simulink model "hopper_6dof_NED_v2_ground"  (R2026a)
settings: Solver=ode3  StopTime=30  FixedStep=1e-3  RelTol=1e-5
undefined symbols (not defined in the file): cg_init, dcg_dMfu_table, dcg_dMox_table, dI_dMfu_table, dI_dMox_table, ENGINE, engine_cg, engine_mass, fu_axial_damping_ratios, fu_lateral_damping_ratios, fu_mass_profile, fu_masses, fu_mdot_data, g, h, IN, K1flat, K2grid, k_leg, m0, magnitude, MoI_init, mount_cg, OUT, ox_axial_damping_ratios, ox_lateral_damping_ratios, ox_mass_profile, ox_masses, ox_mdot_data, pressureLevels, tank_r, TANKS, Target_Trajectory, tgrid, thrust_data, unom, uwndTable, VEH, vwndTable
libraries: fl_lib x31, nesl_utility x25, matrix_library x18, SimscapeFluids_lib x10, simulink x9, simulink_extras x7, slpidlib x7, dspmathops x4, dspindex x3, sl_discontinuities x2, aerolibanim x1, commrandsrc3 x1
(part 7 of 7)

== system hopper_6dof_NED_v2_ground/Wind Forces/If Action Subsystem1 ==
  In1 : Inport
  Action Port : ActionPort  ActionPortLabel=elseif(u1 == 2)
  Constant : Constant  Value=IN.wind.uwind
  Constant1 : Constant  Value=IN.wind.vwind
  Constant3 : Constant  Value=[10;20]
  Mux : Mux  Inputs=2
  Terminator : Terminator
  Out2 : Outport
  wires:
  In1/1 -> Terminator/1
  Mux/1 -> Out2/1
  Constant/1 -> Mux/1
  Constant1/1 -> Mux/2

== system hopper_6dof_NED_v2_ground/Wind Forces/If Action Subsystem2 ==
  In1 : Inport
  Action Port : ActionPort  ActionPortLabel=else
  Display : Display
  Display1 : Display
  Latitude : Constant  Value=33.78
  Longitude : Constant  Value=84.40
  Month : Constant  Value=4
  Mux : Mux  Inputs=2
  Pressure (mb) : Constant  Value=1000
  Terminator : Terminator
  n-D Lookup Table : Lookup_n-D  NumberOfTableDimensions=4  BreakpointsForDimension1=1:12  BreakpointsForDimension2=pressureLevels  BreakpointsForDimension3=[32.5 35]  BreakpointsForDimension4=[82.5 85]  Table=uwndTable  ExtrapMethod=Clip  InternalRulePriority=Speed  RndMeth=Simplest
      settings: InputPortMap=u0,u1,u2,u3
  n-D Lookup Table1 : Lookup_n-D  NumberOfTableDimensions=4  BreakpointsForDimension1=1:12  BreakpointsForDimension2=pressureLevels  BreakpointsForDimension3=[32.5 35]  BreakpointsForDimension4=[82.5 85]  Table=vwndTable  InternalRulePriority=Speed  RndMeth=Simplest
      settings: InputPortMap=u0,u1,u2,u3
  Out1 : Outport
  wires:
  Month/1 -> n-D Lookup Table1/1, n-D Lookup Table/1
  Pressure (mb)/1 -> n-D Lookup Table1/2, n-D Lookup Table/2
  Latitude/1 -> n-D Lookup Table1/3, n-D Lookup Table/3
  In1/1 -> Terminator/1
  Longitude/1 -> n-D Lookup Table1/4, n-D Lookup Table/4
  n-D Lookup Table/1 -> Display/1, Mux/1
  n-D Lookup Table1/1 -> Display1/1, Mux/2
  Mux/1 -> Out1/1

== system hopper_6dof_NED_v2_ground/Fluid Network2/COPV/COPV Leakage ==
  Leak Rate : fl_lib/Gas/Elements/Flow Resistance (G)  delta_p_nominal=0.001 MPa  mdot_nominal=0.0000000001 kg/s  rho_nominal=0 kg/m^3  area=0.01 m^2  laminar_fraction=1e-3
  Mass & Energy Flow Rate Sensor (G)2 : fl_lib/Gas/Sensors/Flow Rate Sensor (G)  mass_flow_measure=true  volumetric_flow_measure=false  volumetric_flow_conditions=foundation.enum.volumetric_flow_conditions.actual  p_std=0.101325 MPa  T_std=20 degC  energy_flow_measure=true
  PS-Simulink Converter7 : nesl_utility/PS-Simulink Converter  PhysicalDomain=network_engine_domain  SubClassName=ps_output  LeftPortType=input  RightPortType=output  PseudoPeriodic=off  Frequencies=[]  VectorFormat=inherit  Unit=inherit  AffineConversion=off
  Pressurant Mass Leak Rate : Scope  Commented=on
      settings: ActiveDisplayYMinimum=-1  ActiveDisplayYMaximum=1
  Reservoir (G) : fl_lib/Gas/Elements/Reservoir (G)  pressure_input=false  pressure_spec=foundation.enum.pressure_spec.atmospheric  reservoir_pressure=0.101325 MPa  temperature_input=false  reservoir_temperature=293.15 K  area_A=0.01 m^2  input_error_spec=foundation.enum.input_range_error.warn
  Conn1 : PMIOPort  Side=Right
  wires:
  PS-Simulink Converter7/1 -> Pressurant Mass Leak Rate/1
  connections:
  Conn1/RConn1 -- Leak Rate/RConn1
  Leak Rate/LConn1 -- Mass & Energy Flow Rate Sensor (G)2/LConn1
  Mass & Energy Flow Rate Sensor (G)2/RConn1 -- Reservoir (G)/LConn1
  Mass & Energy Flow Rate Sensor (G)2/RConn2 -- PS-Simulink Converter7/LConn1

== system hopper_6dof_NED_v2_ground/Ground1/Ground Interaction 1/If Action Subsystem ==
  Velocity : Inport
  Action Port : ActionPort
  Fg : Constant  Value=m0 * IN.const.g0
  Gain : Gain  Gain=-1
  Normalization : dspmathops/Normalization  NormType=Squared 2-norm  Bias=1e-10  NormOver=Each column  Dimension=1  roundingMode=Floor  overflowMode=off  accumDataTypeStr=Inherit: Same as product output  accumLastDataTypeStr=Inherit: Same as product output  outputDataTypeStr=Inherit: Same as product output  outputMin=[]  outputMax=[]  outputLastDataTypeStr=Inherit: Same as product output
  Product : Product  Inputs=3
  mu : Constant  Value=0.6
  Fk : Outport
  wires:
  Velocity/1 -> Normalization/1
  Normalization/1 -> Product/1
  Fg/1 -> Product/2
  mu/1 -> Product/3
  Product/1 -> Gain/1
  Gain/1 -> Fk/1

== system hopper_6dof_NED_v2_ground/Ground1/Ground Interaction 1/If Action Subsystem1 ==
  Action Port : ActionPort
  Zero : Constant  Value=[0 0 0]  OutDataTypeStr=Inherit: Inherit via back propagation
  Out1 : Outport
  wires:
  Zero/1 -> Out1/1

== system hopper_6dof_NED_v2_ground/Ground1/Ground Interaction 2/If Action Subsystem ==
  Velocity : Inport
  Action Port : ActionPort
  Fg : Constant  Value=m0 * IN.const.g0
  Gain : Gain  Gain=-1
  Normalization : dspmathops/Normalization  NormType=Squared 2-norm  Bias=1e-10  NormOver=Each column  Dimension=1  roundingMode=Floor  overflowMode=off  accumDataTypeStr=Inherit: Same as product output  accumLastDataTypeStr=Inherit: Same as product output  outputDataTypeStr=Inherit: Same as product output  outputMin=[]  outputMax=[]  outputLastDataTypeStr=Inherit: Same as product output
  Product : Product  Inputs=3
  mu : Constant  Value=0.6
  Fk : Outport
  wires:
  Velocity/1 -> Normalization/1
  Normalization/1 -> Product/1
  Fg/1 -> Product/2
  mu/1 -> Product/3
  Product/1 -> Gain/1
  Gain/1 -> Fk/1

== system hopper_6dof_NED_v2_ground/Ground1/Ground Interaction 2/If Action Subsystem1 ==
  Action Port : ActionPort
  Zero : Constant  Value=[0 0 0]  OutDataTypeStr=Inherit: Inherit via back propagation
  Out1 : Outport
  wires:
  Zero/1 -> Out1/1

== system hopper_6dof_NED_v2_ground/Ground1/Ground Interaction 3/If Action Subsystem ==
  Velocity : Inport
  Action Port : ActionPort
  Fg : Constant  Value=m0 * IN.const.g0
  Gain : Gain  Gain=-1
  Normalization : dspmathops/Normalization  NormType=Squared 2-norm  Bias=1e-10  NormOver=Each column  Dimension=1  roundingMode=Floor  overflowMode=off  accumDataTypeStr=Inherit: Same as product output  accumLastDataTypeStr=Inherit: Same as product output  outputDataTypeStr=Inherit: Same as product output  outputMin=[]  outputMax=[]  outputLastDataTypeStr=Inherit: Same as product output
  Product : Product  Inputs=3
  mu : Constant  Value=0.6
  Fk : Outport
  wires:
  Velocity/1 -> Normalization/1
  Normalization/1 -> Product/1
  Fg/1 -> Product/2
  mu/1 -> Product/3
  Product/1 -> Gain/1
  Gain/1 -> Fk/1

== system hopper_6dof_NED_v2_ground/Ground1/Ground Interaction 3/If Action Subsystem1 ==
  Action Port : ActionPort
  Zero : Constant  Value=[0 0 0]  OutDataTypeStr=Inherit: Inherit via back propagation
  Out1 : Outport
  wires:
  Zero/1 -> Out1/1

== system hopper_6dof_NED_v2_ground/Ground1/Ground Interaction 4/If Action Subsystem ==
  Velocity : Inport
  Action Port : ActionPort
  Fg : Constant  Value=m0 * IN.const.g0
  Gain : Gain  Gain=-1
  Normalization : dspmathops/Normalization  NormType=Squared 2-norm  Bias=1e-10  NormOver=Each column  Dimension=1  roundingMode=Floor  overflowMode=off  accumDataTypeStr=Inherit: Same as product output  accumLastDataTypeStr=Inherit: Same as product output  outputDataTypeStr=Inherit: Same as product output  outputMin=[]  outputMax=[]  outputLastDataTypeStr=Inherit: Same as product output
  Product : Product  Inputs=3
  mu : Constant  Value=0.6
  Fk : Outport
  wires:
  Velocity/1 -> Normalization/1
  Normalization/1 -> Product/1
  Fg/1 -> Product/2
  mu/1 -> Product/3
  Product/1 -> Gain/1
  Gain/1 -> Fk/1

== system hopper_6dof_NED_v2_ground/Ground1/Ground Interaction 4/If Action Subsystem1 ==
  Action Port : ActionPort
  Zero : Constant  Value=[0 0 0]  OutDataTypeStr=Inherit: Inherit via back propagation
  Out1 : Outport
  wires:
  Zero/1 -> Out1/1

== matlab function hopper_6dof_NED_v2_ground/Slosh/Oxidizer Yaw Force/MATLAB Function ==
  data: ox_yaw_accel input; accel_term output; ox_lateral_pendulum_l input
function accel_term = fcn(ox_yaw_accel, ox_lateral_pendulum_l)

accel_term = -ox_yaw_accel / ox_lateral_pendulum_l;

end

== matlab function hopper_6dof_NED_v2_ground/Slosh/Oxidizer Yaw Force/MATLAB Function1 ==
  data: ox_yaw_phi input; ang_term output; ox_lateral_natural_freq input
function ang_term = fcn(ox_yaw_phi, ox_lateral_natural_freq)

ang_term = -ox_lateral_natural_freq^2 * ox_yaw_phi;

end

== matlab function hopper_6dof_NED_v2_ground/Slosh/Oxidizer Yaw Force/MATLAB Function2 ==
  data: ox_yaw_phi_dot input; velo_term output; ox_lateral_natural_freq input; ox_lateral_damping input
function velo_term = fcn(ox_yaw_phi_dot, ox_lateral_natural_freq,ox_lateral_damping)

velo_term = -2 * ox_lateral_damping * ox_lateral_natural_freq * ox_yaw_phi_dot;
end

== matlab function hopper_6dof_NED_v2_ground/Slosh/Oxidizer Yaw Force/MATLAB Function3 ==
  data: ox_yaw_phi_ddot input; ox_yaw_f output; ox_lateral_slosh_mass input; ox_lateral_pendulum_l input
function ox_yaw_f = fcn(ox_yaw_phi_ddot, ox_lateral_slosh_mass, ox_lateral_pendulum_l)

ox_yaw_f = ox_lateral_slosh_mass * ox_lateral_pendulum_l * ox_yaw_phi_ddot;
end

== matlab function hopper_6dof_NED_v2_ground/Slosh/Oxidizer Axial Force/MATLAB Function ==
  data: ox_axial_accel input; accel_term output; ox_axial_pendulum_l input
function accel_term = fcn(ox_axial_accel, ox_axial_pendulum_l)

accel_term = -ox_axial_accel / ox_axial_pendulum_l;

end

== matlab function hopper_6dof_NED_v2_ground/Slosh/Oxidizer Axial Force/MATLAB Function1 ==
  data: ox_axial_phi input; ang_term output; ox_axial_natural_freq input
function ang_term = fcn(ox_axial_phi, ox_axial_natural_freq)

ang_term = -ox_axial_natural_freq^2 * ox_axial_phi;

end

== matlab function hopper_6dof_NED_v2_ground/Slosh/Oxidizer Axial Force/MATLAB Function2 ==
  data: ox_axial_phi_dot input; velo_term output; ox_axial_natural_freq input; ox_axial_damping input
function velo_term = fcn(ox_axial_phi_dot, ox_axial_natural_freq,ox_axial_damping)

velo_term = -2 * ox_axial_damping * ox_axial_natural_freq * ox_axial_phi_dot;
end

== matlab function hopper_6dof_NED_v2_ground/Slosh/Oxidizer Axial Force/MATLAB Function3 ==
  data: ox_axial_phi_ddot input; ox_axial_f output; ox_axial_slosh_mass input; ox_axial_pendulum_l input
function ox_axial_f = fcn(ox_axial_phi_ddot, ox_axial_slosh_mass, ox_axial_pendulum_l)

ox_axial_f = ox_axial_slosh_mass * ox_axial_pendulum_l * ox_axial_phi_ddot;
end

== matlab function hopper_6dof_NED_v2_ground/Slosh/Fuel Axial Force/MATLAB Function ==
  data: fu_axial_accel input; accel_term output; fu_axial_pendulum_l input
function accel_term = fcn(fu_axial_accel, fu_axial_pendulum_l)

accel_term = -fu_axial_accel / fu_axial_pendulum_l;

end

== matlab function hopper_6dof_NED_v2_ground/Slosh/Fuel Axial Force/MATLAB Function1 ==
  data: fu_axial_phi input; ang_term output; fu_axial_natural_freq input
function ang_term = fcn(fu_axial_phi, fu_axial_natural_freq)

ang_term = -fu_axial_natural_freq^2 * fu_axial_phi;

end

== matlab function hopper_6dof_NED_v2_ground/Slosh/Fuel Axial Force/MATLAB Function2 ==
  data: fu_axial_phi_dot input; velo_term output; fu_axial_natural_freq input; fu_axial_damping input
function velo_term = fcn(fu_axial_phi_dot, fu_axial_natural_freq,fu_axial_damping)

velo_term = -2 * fu_axial_damping * fu_axial_natural_freq * fu_axial_phi_dot;
end

== matlab function hopper_6dof_NED_v2_ground/Slosh/Fuel Axial Force/MATLAB Function3 ==
  data: fu_axial_phi_ddot input; fu_axial_f output; fu_axial_slosh_mass input; fu_axial_pendulum_l input
function fu_axial_f = fcn(fu_axial_phi_ddot, fu_axial_slosh_mass, fu_axial_pendulum_l)

fu_axial_f = fu_axial_slosh_mass * fu_axial_pendulum_l * fu_axial_phi_ddot;
end

== matlab function hopper_6dof_NED_v2_ground/Slosh/Fuel Yaw Force/MATLAB Function ==
  data: fu_pitch_accel input; accel_term output; fu_lateral_pendulum_l input
function accel_term = fcn(fu_pitch_accel, fu_lateral_pendulum_l)

accel_term = -fu_pitch_accel / fu_lateral_pendulum_l;

end

== matlab function hopper_6dof_NED_v2_ground/Slosh/Fuel Yaw Force/MATLAB Function1 ==
  data: fu_pitch_phi input; ang_term output; fu_lateral_natural_freq input
function ang_term = fcn(fu_pitch_phi, fu_lateral_natural_freq)

ang_term = -fu_lateral_natural_freq^2 * fu_pitch_phi;

end

== matlab function hopper_6dof_NED_v2_ground/Slosh/Fuel Yaw Force/MATLAB Function2 ==
  data: fu_pitch_phi_dot input; velo_term output; fu_lateral_natural_freq input; fu_lateral_damping input
function velo_term = fcn(fu_pitch_phi_dot, fu_lateral_natural_freq,fu_lateral_damping)

velo_term = -2 * fu_lateral_damping * fu_lateral_natural_freq * fu_pitch_phi_dot;
end

== matlab function hopper_6dof_NED_v2_ground/Slosh/Fuel Yaw Force/MATLAB Function3 ==
  data: fu_pitch_phi_ddot input; fu_pitch_f output; fu_lateral_slosh_mass input; fu_lateral_pendulum_l input
function fu_pitch_f = fcn(fu_pitch_phi_ddot, fu_lateral_slosh_mass, fu_lateral_pendulum_l)

fu_pitch_f = fu_lateral_slosh_mass * fu_lateral_pendulum_l * fu_pitch_phi_ddot;
end

== matlab function hopper_6dof_NED_v2_ground/Slosh/Fuel Pitch Force/MATLAB Function ==
  data: fu_yaw_accel input; accel_term output; fu_lateral_pendulum_l input
function accel_term = fcn(fu_yaw_accel, fu_lateral_pendulum_l)

accel_term = -fu_yaw_accel / fu_lateral_pendulum_l;

end

== matlab function hopper_6dof_NED_v2_ground/Slosh/MATLAB Function ==
  data: ox_lateral_natural_freq output; ox_axial_natural_freq output; ox_mass input; ox_lateral_slosh_mass output; ox_axial_slosh_mass output; ox_lateral_pendulum_l output; ox_aeff input; ox_axial_pendulum_l output; ox_lateral_damping output; ox_axial_damping output; tank_r input; ox_lateral_damping input; ox_axial_damping input
function [ox_lateral_natural_freq, ox_axial_natural_freq, ox_lateral_slosh_mass,ox_axial_slosh_mass, ox_lateral_pendulum_l, ox_axial_pendulum_l, ox_lateral_damping, ox_axial_damping]  = slosh_parameters(ox_mass, ox_aeff, tank_r, ox_lateral_damping, ox_axial_damping)

zeta = 1.841; % 1st eigen mode of oscillation for a cylindrical tank
ox_density = 1141;   % kg/m^3
% ox_tank_cg = 1.854; % m
% ox_tank_h =  TANKS.singular.oxidizer.h;
geff = norm(ox_aeff) + 0.001;

% Oxidizer Fluid
if ox_mass > 0.001
   h_ox_fluid = (ox_mass / ox_density) / (pi * tank_r^2);

   % Slosh Natural Frequencies
    ox_lateral_natural_freq = sqrt(zeta * geff / tank_r) * tanh(zeta * h_ox_fluid / tank_r);
    ox_axial_natural_freq = pi * sqrt(geff / h_ox_fluid);

    % Slosh Masses 
    ox_lateral_slosh_mass = ox_mass * (2 * tank_r * tanh(2 * zeta * h_ox_fluid / (2 * tank_r))) / (zeta * (zeta^2 - 1) * h_ox_fluid);
    ox_axial_slosh_mass = 1 / (pi^2) *  ox_mass;

    % Slosh Pendulum Lengths
    ox_lateral_pendulum_l = (2 * tank_r) / (2 * zeta * tanh(2*zeta * h_ox_fluid / (2 * tank_r)));
    ox_axial_pendulum_l = geff / ox_axial_natural_freq^2;
else
   h_ox_fluid = 0; 
   ox_lateral_natural_freq = 0;
   ox_axial_natural_freq = 0;
   ox_lateral_slosh_mass = 0;
   ox_axial_slosh_mass = 0;
   ox_lateral_pendulum_l = 1;
   ox_axial_pendulum_l = 1;
end



end

== matlab function hopper_6dof_NED_v2_ground/Slosh/Fuel Pitch Force/MATLAB Function1 ==
  data: fu_yaw_phi input; ang_term output; fu_lateral_natural_freq input
function ang_term = fcn(fu_yaw_phi, fu_lateral_natural_freq)

ang_term = -fu_lateral_natural_freq^2 * fu_yaw_phi;

end

== matlab function hopper_6dof_NED_v2_ground/Slosh/Fuel Pitch Force/MATLAB Function2 ==
  data: fu_yaw_phi_dot input; velo_term output; fu_lateral_natural_freq input; fu_lateral_damping input
function velo_term = fcn(fu_yaw_phi_dot, fu_lateral_natural_freq, fu_lateral_damping)

velo_term = -2 * fu_lateral_damping * fu_lateral_natural_freq * fu_yaw_phi_dot;
end

== matlab function hopper_6dof_NED_v2_ground/Slosh/Fuel Pitch Force/MATLAB Function3 ==
  data: fu_yaw_phi_ddot input; fu_yaw_f output; fu_lateral_slosh_mass input; fu_lateral_pendulum_l input
function fu_yaw_f = fcn(fu_yaw_phi_ddot, fu_lateral_slosh_mass, fu_lateral_pendulum_l)

fu_yaw_f = fu_lateral_slosh_mass * fu_lateral_pendulum_l * fu_yaw_phi_ddot;
end

== matlab function hopper_6dof_NED_v2_ground/CG // MOI Script v3/MATLAB Function ==
  data: r_ox input; I_m_ox output
function I_m_ox = fcn(r_ox)
x = r_ox(1);
y = r_ox(2);
z = r_ox(3);

I_m_ox = [y^2 + z^2 -x*y x*z;
       -x*y x^2 + z^2 -y*z;
       -x*z y*z  x^2 + y^2
    ];

== matlab function hopper_6dof_NED_v2_ground/CG // MOI Script v3/MATLAB Function1 ==
  data: r_fu input; I_m_fu output
function I_m_fu = fcn(r_fu)
x = r_fu(1);
y = r_fu(2);
z = r_fu(3);

I_m_fu = [y^2 + z^2 -x*y x*z;
       -x*y x^2 + z^2 -y*z;
       -x*z y*z  x^2 + y^2
    ];

== matlab function hopper_6dof_NED_v2_ground/Slosh/Oxidizer Axial Force/MATLAB Function4 ==
  data: x_omega_dot input; x_slosh_torque output; ox_axial_slosh_mass input; ox_axial_pendulum_l input; slosh_angular_accel input
function x_slosh_torque = fcn(x_omega_dot, ox_axial_slosh_mass, ox_axial_pendulum_l, slosh_angular_accel)

I_s = ox_axial_slosh_mass * ox_axial_pendulum_l^2;

x_slosh_torque = -I_s*(x_omega_dot - slosh_angular_accel);

== matlab function hopper_6dof_NED_v2_ground/Slosh/Fuel Axial Force/MATLAB Function4 ==
  data: x_omega_dot input; x_slosh_torque output; fu_axial_slosh_mass input; fu_axial_pendulum_l input; slosh_angular_accel input
function x_slosh_torque = fcn(x_omega_dot, fu_axial_slosh_mass, fu_axial_pendulum_l, slosh_angular_accel)

I_s = fu_axial_slosh_mass * fu_axial_pendulum_l^2;

x_slosh_torque = -I_s*(x_omega_dot - slosh_angular_accel);

== matlab function hopper_6dof_NED_v2_ground/Slosh/Oxidizer Yaw Force/MATLAB Function4 ==
  data: y_omega_dot input; y_slosh_torque output; ox_lateral_slosh_mass input; ox_lateral_pendulum_l input; slosh_angular_accel input
function y_slosh_torque = fcn(y_omega_dot, ox_lateral_slosh_mass, ox_lateral_pendulum_l, slosh_angular_accel)

I_s = ox_lateral_slosh_mass * ox_lateral_pendulum_l^2;

y_slosh_torque = -I_s*(y_omega_dot - slosh_angular_accel);

== matlab function hopper_6dof_NED_v2_ground/Slosh/Fuel Yaw Force/MATLAB Function4 ==
  data: y_omega_dot input; y_slosh_torque output; fu_lateral_slosh_mass input; fu_lateral_pendulum_l input; slosh_angular_accel input
function y_slosh_torque = fcn(y_omega_dot, fu_lateral_slosh_mass, fu_lateral_pendulum_l, slosh_angular_accel)

I_s = fu_lateral_slosh_mass * fu_lateral_pendulum_l^2;

y_slosh_torque = -I_s*(y_omega_dot - slosh_angular_accel);

== matlab function hopper_6dof_NED_v2_ground/Slosh/Oxidizer Pitch Force/MATLAB Function4 ==
  data: z_omega_dot input; z_slosh_torque output; ox_lateral_slosh_mass input; ox_lateral_pendulum_l input; slosh_angular_accel input
function z_slosh_torque = fcn(z_omega_dot, ox_lateral_slosh_mass, ox_lateral_pendulum_l, slosh_angular_accel)

I_s = ox_lateral_slosh_mass * ox_lateral_pendulum_l^2;

z_slosh_torque = -I_s*(z_omega_dot - slosh_angular_accel);

== matlab function hopper_6dof_NED_v2_ground/Slosh/Fuel Pitch Force/MATLAB Function4 ==
  data: z_omega_dot input; z_slosh_torque output; fu_lateral_slosh_mass input; fu_lateral_pendulum_l input; slosh_angular_accel input
function z_slosh_torque = fcn(z_omega_dot, fu_lateral_slosh_mass, fu_lateral_pendulum_l, slosh_angular_accel)

I_s = fu_lateral_slosh_mass * fu_lateral_pendulum_l^2;

z_slosh_torque = -I_s*(z_omega_dot - slosh_angular_accel);

== matlab function hopper_6dof_NED_v2_ground/CG // MOI Script v3/MATLAB Function2 ==
  data: delta_y input; rot_mat output; delta_z input
function rot_mat = fcn(delta_y, delta_z)

rot_mat = [0 -delta_z delta_y;
           delta_z 0 0;
           -delta_y 0 0];

== matlab function hopper_6dof_NED_v2_ground/Fluid Network2/Fuel Throttle Valve Controller/Feed Forward ==
  data: mdot input; theta output; ptank input; pset input; rho input; CdA output
function [theta, CdA] = feed_forward(mdot,ptank,pset,rho)

dp = max(ptank - pset, 1e-6); % divide by zero error
CdA = mdot / sqrt(2*dp*rho);

CdA = max(CdA, 1e-7); % divide by zero error
Cv_vector = [1e-8, 0.01, 0.06, 0.21, 0.46, 0.83, 1.35, 2.04, 2.93];
CdA_vector = Cv_vector ./ 37.97;
theta_vector = 0.9.*[20,30,40,50,60,70,80,90,100];

theta = interp1(CdA_vector, theta_vector, CdA);
theta = min(theta, 90);
theta = max(theta, 0);
end

== matlab function hopper_6dof_NED_v2_ground/Fluid Network2/Fuel Throttle Valve Controller/MATLAB Function5 ==
  data: time input; rate_limit_up output; rate_limit_down output
function [rate_limit_up, rate_limit_down] = fcn(time)
if time < 0.5
    rate_limit_up = 1350;
else
    rate_limit_up = 40;
end
rate_limit_down = -rate_limit_up;

== matlab function hopper_6dof_NED_v2_ground/Fluid Network2/Fuel Throttle Valve Controller/System ==
  data: Ptank input; CdA input; mdot input; Pout output; rho input; dp output
function [Pout,dp] = theta_to_pressure(Ptank,CdA,mdot, rho)

% CdA = mdot/(sqrt((2*(ptank-pout)*rho)

%CdA = max(CdA, 1e-7);
dp = (mdot/CdA)^2*1/(2*rho);

% (mdot/CdA)^2*rho/2 is solving for the pout from the dp in CdA eqn
Pout = Ptank - dp;
Pout = max(Pout, 0);

== matlab function hopper_6dof_NED_v2_ground/Fluid Network2/MATLAB Function ==
  data: mdot_ox input; mdot_fuel input; eta_cstar input; Cf input; thrust output; Pc output; MR output; cstar_ideal input
function [thrust, Pc, MR] = engine_model(mdot_ox, mdot_fuel, eta_cstar, Cf, cstar_ideal)
%#codegen
% ENGINE_MODEL
%
% Inputs:
%   mdot_ox      - oxidizer mass flow rate [kg/s]
%   mdot_fuel    - fuel mass flow rate [kg/s]
%   eta_cstar    - c* efficiency [-]
%   Cf           - thrust coefficient [-]
%
% Outputs:
%   thrust       - thrust [N]
%   Pc           - chamber pressure [Pa]
%   MR           - mixture ratio [-]

    %% -------------------------
    % CONSTANTS
    % -------------------------
    At = 0.0008271;      % throat area [m^2]

    %% -------------------------
    % 1. Total mass flow
    % -------------------------
    mdot = mdot_ox + mdot_fuel;

    %% -------------------------
    % 2. Mixture ratio
    % -------------------------
    if mdot_fuel > 0
        MR = mdot_ox / mdot_fuel;
    else
        MR = 0; % avoid divide by zero
    end

    %% -------------------------
    % 3. Actual c*
    % -------------------------
    cstar_actual = eta_cstar * cstar_ideal;

    %% -------------------------
    % 4. Chamber pressure
    % -------------------------
    Pc = (mdot * cstar_actual) / At;

    %% -------------------------
    % 6. Thrust
    % -------------------------
    thrust = Cf * Pc * At;

    % Equivalent:
    % thrust = Cf * mdot * cstar_actual;

end

== matlab function hopper_6dof_NED_v2_ground/Fluid Network2/Ox Throttle Valve Controller/Feed Forward ==
  data: mdot input; theta output; ptank input; pset input; rho input; CdA output
function [theta, CdA] = feed_forward(mdot,ptank,pset,rho)

dp = max(ptank - pset, 1e-6); % divide by zero error
CdA = mdot / sqrt(2*dp*rho);

CdA = max(CdA, 1e-7); % divide by zero error
Cv_vector = [1e-8, 0.01, 0.06, 0.21, 0.46, 0.83, 1.35, 2.04, 2.93];
CdA_vector = Cv_vector ./ 37.97;
theta_vector = 0.9.*[20,30,40,50,60,70,80,90,100];

theta = interp1(CdA_vector, theta_vector, CdA);
theta = min(theta, 90);
theta = max(theta, 0);
end

== matlab function hopper_6dof_NED_v2_ground/Fluid Network2/Ox Throttle Valve Controller/MATLAB Function5 ==
  data: time input; rate_limit_up output; rate_limit_down output
function [rate_limit_up, rate_limit_down] = fcn(time)
if time < 0.5
    rate_limit_up = 1350;
else
    rate_limit_up = 40;
end
rate_limit_down = -rate_limit_up;

== matlab function hopper_6dof_NED_v2_ground/Fluid Network2/Ox Throttle Valve Controller/System ==
  data: Ptank input; CdA input; mdot input; Pout output; rho input; dp output
function [Pout,dp] = theta_to_pressure(Ptank,CdA,mdot, rho)

% CdA = mdot/(sqrt((2*(ptank-pout)*rho)

%CdA = max(CdA, 1e-7);
dp = (mdot/CdA)^2*1/(2*rho);

% (mdot/CdA)^2*rho/2 is solving for the pout from the dp in CdA eqn
Pout = Ptank - dp;
Pout = max(Pout, 0);

== matlab function hopper_6dof_NED_v2_ground/MATLAB Function ==
  data: t input; u output; x input; tgrid input; xref input; K1flat input; K2grid input; unom input
function u = Gain_Selector(t, x, tgrid, xref, K1flat, K2grid, unom)
%#codegen
% Fixed-size output: u is always 4x1

u = zeros(4,1);

x = x(:);              % should be 13x1 for 6DOF
N = length(tgrid);

% --- Clamp time and compute interval index ---
if t <= tgrid(1)
    idx = 1;
    w = 0.0;
elseif t >= tgrid(end)
    idx = N-1;
    w = 1.0;
else
    idx = 1;
    for k = 1:(N-1)
        if tgrid(k) <= t && t < tgrid(k+1)
            idx = k;
            break;
        end
    end
    t1 = tgrid(idx);
    t2 = tgrid(idx+1);
    w  = (t - t1) / (t2 - t1);
end

% --- Interpolate reference state (13x1) ---
xref_t = (1-w)*xref(idx,:)' + w*xref(idx+1,:)';

% --- Interpolate K1flat then reshape to 4x13 ---
Kflat = (1-w)*K1flat(idx,:) + w*K1flat(idx+1,:);
K1 = reshape(Kflat, 13, 4)';   % 4x13   (requires K1flat is N×52)

% --- Interpolate K2 (4x1) ---
K2 = (1-w)*K2grid(idx,:)' + w*K2grid(idx+1,:)';

% --- Interpolate nominal control (4x1) ---
u_nom = (1-w)*unom(idx,:)' + w*unom(idx+1,:)';

q     = x(10:13);
qref  = xref_t(10:13);

if dot(q,qref) < 0
    q = -q;
end

x_used = x;
x_used(10:13) = q;

dx = x_used - xref_t;


% --- Control law ---
%dx = (x - xref_t);          % 13x1
u  =u_nom+(-K1*dx)-K2;  
%fix

end

== matlab function hopper_6dof_NED_v2_ground/Fluid Network2/Thrust Commanded to mdot + bunch of other bs ==
  data: mdot_fuel output; rho_fuel_eng output; pc output; F_cmd input; rho_ox input; rho_fuel input; rho_ox_eng output; mdot_ox output; Cf input; MR input; cstar_ideal input; cstar_eff input
function [mdot_fuel, rho_fuel_eng, pc, rho_ox_eng, mdot_ox] = thrust_to_mdot( ...
   F_cmd, rho_ox, rho_fuel, Cf, MR, cstar_ideal, cstar_eff)
%#codegen
% Convert commanded thrust into mdots and convert densities to English units
%
% Outputs:
%   mdot_ox        - oxidizer mass flow rate [kg/s]
%   mdot_fuel      - fuel mass flow rate [kg/s]
%   rho_ox_eng     - oxidizer density [lb/ft^3]
%   rho_fuel_eng   - fuel density [lb/ft^3]
%   mdot_ox_lb     - oxidizer mass flow rate [lb/s]
%   mdot_fuel_lb   - fuel mass flow rate [lb/s]

    cstar = cstar_ideal * cstar_eff;
    At = 0.0008271;      % throat area [m^2]

    %% ---- DEFAULT OUTPUTS ----
    mdot_ox = 0;
    mdot_fuel = 0;
    rho_ox_eng = 0;
    rho_fuel_eng = 0;
    mdot_ox_lb = 0;
    mdot_fuel_lb = 0;

    %% ---- UNIT CONVERSION ----
    kgm3_to_lbft3 = 0.062428;
    kg_to_lb = 2.20462;

    rho_ox_eng = rho_ox * kgm3_to_lbft3;
    rho_fuel_eng = rho_fuel * kgm3_to_lbft3;

    %% ---- EFFECTIVE EXHAUST VELOCITY ----
    ve = Cf * cstar;


    %% ---- TOTAL MASS FLOW ----
    mdot_total = F_cmd / ve;

    pc = mdot_total * cstar / At;

    pc = pc * 0.000145038;

    %% ---- SPLIT BY MR ----
    mdot_ox = mdot_total * MR / (1 + MR);
    mdot_fuel = mdot_total / (1 + MR);


end

== matlab function hopper_6dof_NED_v2_ground/Slosh/MATLAB Function1 ==
  data: fu_mass input; fu_lateral_natural_freq output; fu_axial_natural_freq output; fu_lateral_slosh_mass output; fu_aeff input; fu_axial_slosh_mass output; fu_lateral_pendulum_l output; fu_axial_pendulum_l output; fu_lateral_damping output; fu_axial_damping output; tank_r input; fu_lateral_damping input; fu_axial_damping input
function [fu_lateral_natural_freq, fu_axial_natural_freq, fu_lateral_slosh_mass, fu_axial_slosh_mass, fu_lateral_pendulum_l, fu_axial_pendulum_l, fu_lateral_damping, fu_axial_damping]  = slosh_parameters(fu_mass, fu_aeff, tank_r, fu_lateral_damping, fu_axial_damping) 
zeta = 1.841; % 1st eigen mode of oscillation for a cylindrical tank
fu_density = 800;    % kg/m^3
% fu_tank_cg = 1.0668; % m
% fu_tank_h = TANKS.singular.fuel.h;
geff = norm(fu_aeff) + 0.001;

if fu_mass > 0.001
   h_fu_fluid = (fu_mass / fu_density) / (pi * tank_r^2);
   % Fluid sits at the bottom of the tank shell
   % z_fu_fluid = (fu_tank_cg - fu_tank_h/2) + (h_fu_fluid / 2);

   % Slosh Natural Frequencies
    fu_lateral_natural_freq = sqrt(zeta * geff / tank_r) * tanh(zeta * h_fu_fluid / tank_r);
    fu_axial_natural_freq = pi * sqrt(geff / h_fu_fluid);

    % Slosh Masses 
    fu_lateral_slosh_mass = fu_mass * (2 * tank_r * tanh(2 * zeta * h_fu_fluid / (2 * tank_r))) / (zeta * (zeta^2 - 1) * h_fu_fluid);
    fu_axial_slosh_mass = 1 / (pi^2) *  fu_mass;

    % Slosh Pendulum Lengths
    fu_lateral_pendulum_l = (2 * tank_r) / (2 * zeta * tanh(2*zeta * h_fu_fluid / (2 * tank_r)));
    fu_axial_pendulum_l = geff / fu_axial_natural_freq^2;
else
   h_fu_fluid = 0;
   fu_lateral_natural_freq = 0;
   fu_axial_natural_freq = 0;
   fu_lateral_slosh_mass = 0;
   fu_axial_slosh_mass = 0;
   fu_lateral_pendulum_l = 1;
   fu_axial_pendulum_l = 1;
end





end

== matlab function hopper_6dof_NED_v2_ground/Slosh/Oxidizer Pitch Force/MATLAB Function ==
  data: ox_pitch_accel input; accel_term output; ox_lateral_pendulum_l input
function accel_term = fcn(ox_pitch_accel, ox_lateral_pendulum_l)

accel_term = -ox_pitch_accel / ox_lateral_pendulum_l;

end

== matlab function hopper_6dof_NED_v2_ground/Slosh/Oxidizer Pitch Force/MATLAB Function1 ==
  data: ox_pitch_phi input; ang_term output; ox_lateral_natural_freq input
function ang_term = fcn(ox_pitch_phi, ox_lateral_natural_freq)

ang_term = -ox_lateral_natural_freq^2 * ox_pitch_phi;

end

== matlab function hopper_6dof_NED_v2_ground/Slosh/Oxidizer Pitch Force/MATLAB Function2 ==
  data: ox_pitch_phi_dot input; velo_term output; ox_lateral_natural_freq input; ox_lateral_damping input
function velo_term = fcn(ox_pitch_phi_dot, ox_lateral_natural_freq,ox_lateral_damping)

velo_term = -2 * ox_lateral_damping * ox_lateral_natural_freq * ox_pitch_phi_dot;
end

== matlab function hopper_6dof_NED_v2_ground/Slosh/Oxidizer Pitch Force/MATLAB Function3 ==
  data: ox_pitch_phi_ddot input; ox_pitch_f output; ox_lateral_slosh_mass input; ox_lateral_pendulum_l input
function ox_pitch_f = fcn(ox_pitch_phi_ddot, ox_lateral_slosh_mass, ox_lateral_pendulum_l)

ox_pitch_f = ox_lateral_slosh_mass * ox_lateral_pendulum_l * ox_pitch_phi_ddot;
end
